simulink model "room207_demo"  (R2026b)
settings: Solver=ode15s  StopTime=inf  RelTol=1e-6  AbsTol=1e-8
PreLoadFcn:
  | if exist('room207_setup', 'file'), room207_setup(); end
StartFcn:
  | room207.viewer('start', bdroot, {'Simulink LIMO'});
StopFcn:
  | room207.viewer('stop');
libraries: limo_lib x1
settings Model: Creator=jkreiss  LastModifiedBy=jkreiss
settings DataIOCC: SaveOutput=off  SaveTime=off

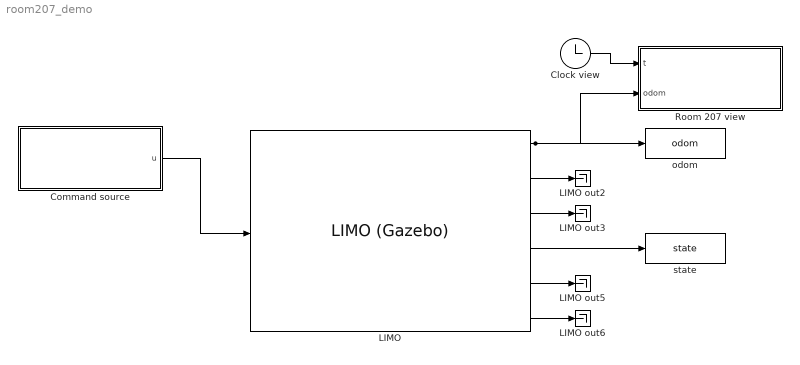
== system room207_demo ==
  Clock view : Clock
  Command source : Subsystem
  LIMO : limo_lib/LIMO (Gazebo)  input_mode=Steering angle: [v; gamma]  pose_mode=Room 207 spawn  custom_pose=[0 0 0]  mu=1  v_eps=1e-3
      settings: SourceProductName=LIMO (ENSEM)
  LIMO out{2..3,5..6} (4 alike) : Terminator
  Room 207 view : MATLAB Function  TreatAsAtomicUnit=on  SystemSampleTime=0.05
  odom : ToWorkspace  VariableName=odom  SaveFormat=Timeseries  SampleTime=-1
  state : ToWorkspace  VariableName=state  SaveFormat=Timeseries  SampleTime=-1
  wires:
  Command source/1(u) -> LIMO/1
  Clock view/1 -> Room 207 view/1(t)
  LIMO/1 -> Room 207 view/2(odom), odom/1
  LIMO/4 -> state/1
  LIMO/2 -> LIMO out2/1
  LIMO/3 -> LIMO out3/1
  LIMO/5 -> LIMO out5/1
  LIMO/6 -> LIMO out6/1

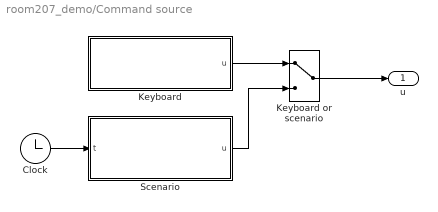
== system room207_demo/Command source ==
  Clock : Clock
  Keyboard : MATLAB Function  TreatAsAtomicUnit=on  SystemSampleTime=0.05
  Keyboard or scenario : ManualSwitch
  Scenario : MATLAB Function  TreatAsAtomicUnit=on
  u : Outport
  wires:
  Scenario/1(u) -> Keyboard or scenario/2
  Clock/1 -> Scenario/1(t)
  Keyboard/1(u) -> Keyboard or scenario/1
  Keyboard or scenario/1 -> u/1

== matlab function room207_demo/Command source/Keyboard ==
  data: u output
function u = keyboard_command()
%KEYBOARD_COMMAND [v; gamma] from the keyboard (room207.viewer).
%   Z/S: forward/backward, Q/D: left/right, Space: stop, Esc: end.

coder.extrinsic('room207.viewer');

u = zeros(2, 1);
u = room207.viewer('command');

== matlab function room207_demo/Room 207 view ==
  data: t input; odom input
function view(t, odom)
%VIEW Draw the LIMO on the Room 207 track (room207.viewer).

coder.extrinsic('room207.viewer');

room207.viewer('draw', t, odom(1:3));

== matlab function room207_demo/Command source/Scenario ==
  data: t input; u output
function u = scenario(t)
%SCENARIO Speed and steering angle as a function of time.
%   u = [v (m/s); gamma (rad)], gamma > 0 to the left
%
%   From the Room 207 spawn: leave the parking bay, turn left into the
%   car park, stop, then reverse along the same arc back into the bay.

v = 0;
gamma = 0;

if t >= 1 && t < 7.3
    v = 0.3;
elseif t >= 8 && t < 14.3
    v = -0.3;
end

if (t >= 4.3 && t < 7.3) || (t >= 8 && t < 11)
    gamma = 0.35;
end

u = [v; gamma];
